simulink model "AXU5EV_Motor_Control_System"  (R2026b)
settings: Solver=FixedStepDiscrete  StopTime=0.1
model workspace (MAT data in the model file):
  ADC_Calibration_Log2_N = 10
  ADC_Manual_Offset_Valid_A = 0
  ADC_Manual_Offset_Valid_B = 0
  Angle_Init_EN : Simulink.Signal (value not decoded)
  Encoder_Counts_Per_Electrical_Period = 30000
  Encoder_Nanometres_Per_Count = 1000
  Experiment_Id_Limit_A = 0.5
  Experiment_Iq_Limit_A = 0.3
  Experiment_Parameter_Version = 20261117
  FOC_Fixed_Config : object (value not decoded)
  FOC_Fixed_Parameters : object (value not decoded)
  Feedback_Id_Step = 500
  Feedback_Tick_Hz = 50000000
  Feedback_Tick_Step = 5000
  Grating_Resolution_mm_per_count = 0.001
  Hardware_Binding_Complete = 0
  Hold_Ticks = 30000
  Host_AutoStart_EN = 0
  Host_Load_N = 0
  Host_Ready_Ticks = 5
  Host_Speed_Ramp_s = 0.2
  Host_Start_s = 0.05
  Host_Traj_Amax = 200
  Host_Traj_Jmax = 1000
  Host_Traj_Vmax = 20
  Id_Init_Step = 5e-05
  Id_Init_Target = 0.5
  Id_Release_Ramp_Ticks = 2000
  Init_Done : Simulink.Signal (value not decoded)
  Init_State_Num : Simulink.Signal (value not decoded)
  Iq_fric_run = 0.05
  Iq_fric_start = 0.4
  Iq_int_limit = 0.2
  Kaw_d = 0.0122881355932
  Kaw_q = 0.0122881355932
  Kaw_s = 0.4
  Ki_ACR = 7250
  Ki_ASR = 0.05
  Kp_ACR = 59
  Kp_ASR = 0.03
  Kp_pos = 5
  PMLSM_Kf_peak_N_per_Apeak = 21.4960461481
  PMLSM_Ld_H = 0.0118
  PMLSM_Lq_H = 0.0118
  PMLSM_Rs_ohm = 1.45
  PMLSM_psi_f_Wb = 0.0684240400279
  PMLSM_tau_NN_m = 0.03
  Physical_Calibration_Valid = 0
  Pos_deadband = 0.02
  Ramp_Ticks = 10000
  Speed_loop_Iq_Limit = 0.3
  Tau_e_mm = 30
  Theta_Offset_Fine = 0
  Theta_Offset_auto : Simulink.Signal (value not decoded)
  Total_Moving_Mass_Known = 0
  Total_Moving_Mass_kg = nan
  Ts = 0.0001
  Ts_ACR = 0.0001
  Ts_ASR = 0.001
  Ts_POS = 0.01
  Tuning_Current_Xi = 0.707106781187
  Udc = 48
  V_meas_max = 500
  V_pos_max_mmps = 20
  X_max_hard = 120
  X_max_soft = 110
  X_min_hard = -120
  X_min_soft = -110
  delay_N = 50
  id_init_ref : Simulink.Signal (value not decoded)
  theta_align_const = 0
  v_ff_eps = 0.5
  v_meas_zero_eps = 0.5
  v_over_eps = 3
  v_ref_max = 20
  v_ref_set_rate_dn = 100
  v_ref_set_rate_up = 100
  v_ref_set_step_dn = 0.01
  v_ref_set_step_up = 0.01
  v_ref_zero_eps = 0
  x_align_mm_latch : Simulink.Signal (value not decoded)
undefined symbols (not defined in the file): v_stick_off, v_stick_on
libraries: simulink x8
(part 2 of 2)

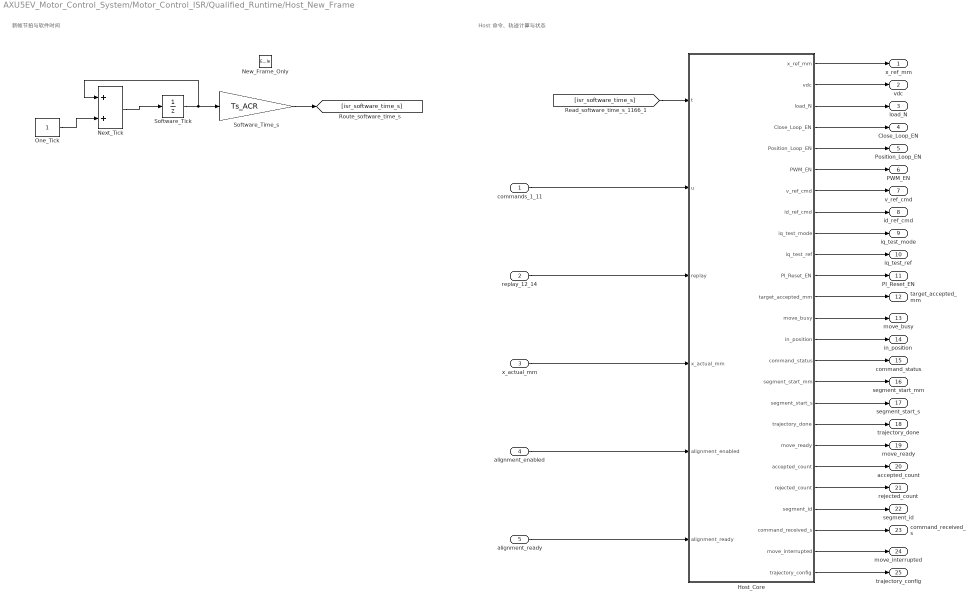
== system AXU5EV_Motor_Control_System/Motor_Control_ISR/Qualified_Runtime/Host_New_Frame ==
  note: 新帧节拍与软件时间
  note: Host 命令、轨迹计算与状态
  commands_1_11 : Inport
  replay_12_14 : Inport  Port=2
  x_actual_mm : Inport  Port=3
  alignment_enabled : Inport  Port=4
  alignment_ready : Inport  Port=5
  New_Frame_Only : EnablePort
  Host_Core : MATLAB Function  TreatAsAtomicUnit=on
  Next_Tick : Sum
  One_Tick : Constant  SampleTime=-1
  Software_Tick : UnitDelay  SampleTime=-1
  Software_Time_s : Gain  Gain=Ts_ACR
  x_ref_mm : Outport
  vdc : Outport  Port=2
  load_N : Outport  Port=3
  Close_Loop_EN : Outport  Port=4
  Position_Loop_EN : Outport  Port=5
  PWM_EN : Outport  Port=6
  v_ref_cmd : Outport  Port=7
  id_ref_cmd : Outport  Port=8
  iq_test_mode : Outport  Port=9
  iq_test_ref : Outport  Port=10
  PI_Reset_EN : Outport  Port=11
  target_accepted_mm : Outport  Port=12
  move_busy : Outport  Port=13
  in_position : Outport  Port=14
  command_status : Outport  Port=15
  segment_start_mm : Outport  Port=16
  segment_start_s : Outport  Port=17
  trajectory_done : Outport  Port=18
  move_ready : Outport  Port=19
  accepted_count : Outport  Port=20
  rejected_count : Outport  Port=21
  segment_id : Outport  Port=22
  command_received_s : Outport  Port=23
  move_interrupted : Outport  Port=24
  trajectory_config : Outport  Port=25
  wires:
  Host_Core/24(move_interrupted) -> move_interrupted/1
  Host_Core/23(command_received_s) -> command_received_s/1
  Host_Core/19(move_ready) -> move_ready/1
  Host_Core/18(trajectory_done) -> trajectory_done/1
  Host_Core/21(rejected_count) -> rejected_count/1
  x_actual_mm/1 -> Host_Core/4(x_actual_mm)
  Host_Core/22(segment_id) -> segment_id/1
  Host_Core/14(in_position) -> in_position/1
  Host_Core/13(move_busy) -> move_busy/1
  alignment_enabled/1 -> Host_Core/5(alignment_enabled)
  Host_Core/12(target_accepted_mm) -> target_accepted_mm/1
  Host_Core/9(iq_test_mode) -> iq_test_mode/1
  replay_12_14/1 -> Host_Core/3(replay)
  Host_Core/11(PI_Reset_EN) -> PI_Reset_EN/1
  Host_Core/7(v_ref_cmd) -> v_ref_cmd/1
  commands_1_11/1 -> Host_Core/2(u)
  Host_Core/10(iq_test_ref) -> iq_test_ref/1
  Host_Core/6(PWM_EN) -> PWM_EN/1
  Host_Core/5(Position_Loop_EN) -> Position_Loop_EN/1
  Host_Core/4(Close_Loop_EN) -> Close_Loop_EN/1
  Host_Core/8(id_ref_cmd) -> id_ref_cmd/1
  Host_Core/16(segment_start_mm) -> segment_start_mm/1
  One_Tick/1 -> Next_Tick/2
  Host_Core/1(x_ref_mm) -> x_ref_mm/1
  Next_Tick/1 -> Software_Tick/1
  Host_Core/3(load_N) -> load_N/1
  Host_Core/25(trajectory_config) -> trajectory_config/1
  Host_Core/17(segment_start_s) -> segment_start_s/1
  Host_Core/15(command_status) -> command_status/1
  Host_Core/20(accepted_count) -> accepted_count/1
  Host_Core/2(vdc) -> vdc/1
  alignment_ready/1 -> Host_Core/6(alignment_ready)
  Software_Tick/1 -> Software_Time_s/1, Next_Tick/1
  [isr_software_time_s] -> Host_Core/1(t)
  Software_Time_s/1 -> [isr_software_time_s]

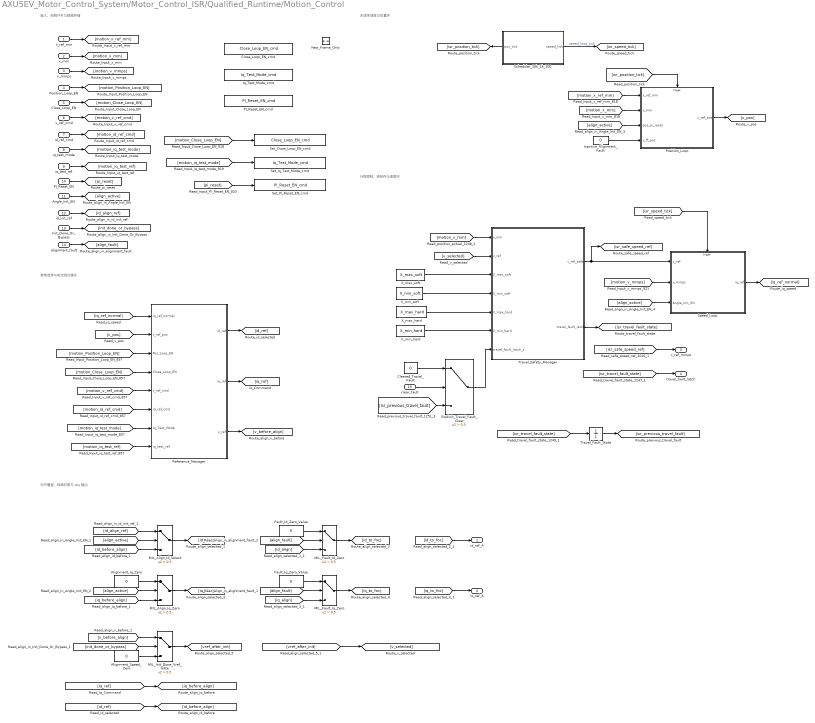
== system AXU5EV_Motor_Control_System/Motor_Control_ISR/Qualified_Runtime/Motion_Control ==
  note: 输入、控制许可与数据存储
  note: 多速率调度与位置环
  note: 参考选择与电流测试模式
  note: 行程限制、清锁存与速度环
  note: 对齐覆盖、故障归零与 d/q 输出
  x_ref_mm : Inport
  x_mm : Inport  Port=2
  v_mmps : Inport  Port=3
  Position_Loop_EN : Inport  Port=4
  Close_Loop_EN : Inport  Port=5
  v_ref_cmd : Inport  Port=6
  id_ref_cmd : Inport  Port=7
  iq_test_mode : Inport  Port=8
  iq_test_ref : Inport  Port=9
  PI_Reset_EN : Inport  Port=10
  Angle_Init_EN : Inport  Port=11
  id_init_ref : Inport  Port=12
  Init_Done_Or_Bypass : Inport  Port=13
  alignment_fault : Inport  Port=14
  clear_fault : Inport  Port=15  OutDataTypeStr=boolean  PortDimensions=1
  New_Frame_Only : EnablePort
  Alignment_Iq_Zero : Constant  Value=0  OutDataTypeStr=double
  Alignment_Speed_Zero : Constant  Value=0  OutDataTypeStr=double
  Cleared_Travel_Fault : Constant  Value=0  OutDataTypeStr=double
  Close_Loop_EN_cmd : DataStoreMemory  DataStoreName=Close_Loop_EN_cmd  WriteAfterWriteMsg=warning  InitialValue=1  ShowAdditionalParam=off
  Explicit_Travel_Fault_Clear : Switch  Criteria=u2 > Threshold  Threshold=0.5  SaturateOnIntegerOverflow=off  InputSameDT=off
  Fault_Id_Zero_Value : Constant  Value=0  OutDataTypeStr=double
  Fault_Iq_Zero_Value : Constant  Value=0  OutDataTypeStr=double
  Inactive_Alignment_Fault : Constant  Value=0
  Iq_Test_Mode_cmd : DataStoreMemory  DataStoreName=Iq_Test_Mode_cmd  WriteAfterWriteMsg=warning  ShowAdditionalParam=off
  MIL_Align_Id_Select : Switch  Criteria=u2 > Threshold  Threshold=0.5  SaturateOnIntegerOverflow=off  InputSameDT=off
  MIL_Align_Iq_Zero : Switch  Criteria=u2 > Threshold  Threshold=0.5  SaturateOnIntegerOverflow=off  InputSameDT=off
  MIL_Fault_Id_Zero : Switch  Criteria=u2 > Threshold  Threshold=0.5  SaturateOnIntegerOverflow=off  InputSameDT=off
  MIL_Fault_Iq_Zero : Switch  Criteria=u2 > Threshold  Threshold=0.5  SaturateOnIntegerOverflow=off  InputSameDT=off
  MIL_Init_Done_Vref_Gate : Switch  Criteria=u2 > Threshold  Threshold=0.5  SaturateOnIntegerOverflow=off  InputSameDT=off
  PI_Reset_EN_cmd : DataStoreMemory  DataStoreName=PI_Reset_EN_cmd  WriteAfterWriteMsg=warning  ShowAdditionalParam=off
  Position_Loop : Subsystem  TreatAsAtomicUnit=on
  Reference_Manager : Subsystem
  Scheduler_10k_1k_100 : Subsystem
      settings: PortSchema="{\"entries\":[{\"content\":{\"sides\":[{\"content\":{\"connectorIds\":[\"Out2\"]},\"type\":\"ConnectorPlacement.EquallySpacedRectSide\",\"uuid\":\"7a2cd2ad-1b6d-4ced-b4c0-dea2e76e4441\"},{\"content\":{\"connectorIds\":[\"Out1\"],\"side\":\"RIGHT\"},\"type\":\"ConnectorPlacement.EquallySpacedRectSide\",\"uuid\":\"f7db3b94-1126-4089-83bd-8e57d20e6fd7\"},{\"content\":{\"side\":\"TOP\"},\"type\":\"ConnectorPlacement.EquallySpacedRectSide\",\"uuid\":\"9153f6b5-22af-48be-92c0-68be43f93648\"}]},\"type\":\"ConnectorPlacement.EquallySpacedConnector\",\"uuid\":\"029fb485-bddc-4cd2-9c64-7547c8dffd2b\"}],\"packageUris\":[\"http://schema.mathworks.com/mf0/Connector/R2020b\"],\"version\":\"1.0\"}"
  Set_Close_Loop_EN_cmd : DataStoreWrite  Priority=-10  DataStoreName=Close_Loop_EN_cmd  IndexOptions=Index vector (dialog)  Indices=1  OutputSizes=1
  Set_Iq_Test_Mode_cmd : DataStoreWrite  Priority=-10  DataStoreName=Iq_Test_Mode_cmd  IndexOptions=Index vector (dialog)  Indices=1  OutputSizes=1
  Set_PI_Reset_EN_cmd : DataStoreWrite  Priority=-10  DataStoreName=PI_Reset_EN_cmd  IndexOptions=Index vector (dialog)  Indices=1  OutputSizes=1
  Speed_Loop : Subsystem  TreatAsAtomicUnit=on
  Travel_Fault_State : UnitDelay  SampleTime=-1
  Travel_Safety_Manager : MATLAB Function  Description=Soft +/-110 mm acts on the final speed reference before Speed_Loop and permits inward motion. Direct Iq test does not share this soft-speed limiting path. Hard +/-120 mm inclusive latches until qualified explicit clear. Mechanical encoder origin is independent of the electrical alignment offset.  TreatAsAtomicUnit=on
  X_max_hard : Constant  Value=X_max_hard  OutDataTypeStr=double
  X_max_soft : Constant  Value=X_max_soft  OutDataTypeStr=double
  X_min_hard : Constant  Value=X_min_hard  OutDataTypeStr=double
  X_min_soft : Constant  Value=X_min_soft  OutDataTypeStr=double
  id_ref_A : Outport
  iq_ref_A : Outport  Port=2
  v_ref_mmps : Outport  Port=3
  travel_fault_latch : Outport  Port=4  OutDataTypeStr=double  PortDimensions=1
  wires:
  [iq_to_foc] -> iq_ref_A/1
  [id_to_foc] -> id_ref_A/1
  [iq_ref_normal] -> Reference_Manager/1(iq_ref_normal)
  [v_pos] -> Reference_Manager/2(v_ref_pos)
  Inactive_Alignment_Fault/1 -> Position_Loop/4(v_ff_pos)
  Position_Loop/1(v_ref_pos) -> [v_pos]
  Reference_Manager/1(id_ref) -> [id_ref]
  Reference_Manager/2(iq_ref) -> [iq_ref]
  MIL_Align_Id_Select/1 -> [id_align]
  [id_align] -> MIL_Fault_Id_Zero/3
  MIL_Fault_Id_Zero/1 -> [id_to_foc]
  MIL_Align_Iq_Zero/1 -> [iq_align]
  [iq_align] -> MIL_Fault_Iq_Zero/3
  MIL_Fault_Iq_Zero/1 -> [iq_to_foc]
  [vref_after_init] -> [v_selected]
  Angle_Init_EN/1 -> [align_active]
  [align_active] -> Position_Loop/3(pos_pi_reset)
  id_init_ref/1 -> [id_align_ref]
  Init_Done_Or_Bypass/1 -> [init_done_or_bypass]
  alignment_fault/1 -> [align_fault]
  [align_fault] -> MIL_Fault_Iq_Zero/2
  [align_fault] -> MIL_Fault_Id_Zero/2
  [id_ref] -> [id_before_align]
  [id_before_align] -> MIL_Align_Id_Select/3
  [iq_ref] -> [iq_before_align]
  [iq_before_align] -> MIL_Align_Iq_Zero/3
  Reference_Manager/3(v_ref) -> [v_before_align]
  [pi_reset] -> Set_PI_Reset_EN_cmd/1
  iq_test_ref/1 -> [motion_iq_test_ref]
  [motion_iq_test_ref] -> Reference_Manager/8(iq_test_ref)
  iq_test_mode/1 -> [motion_iq_test_mode]
  [motion_iq_test_mode] -> Reference_Manager/7(Iq_Test_Mode)
  [motion_iq_test_mode] -> Set_Iq_Test_Mode_cmd/1
  id_ref_cmd/1 -> [motion_id_ref_cmd]
  [motion_id_ref_cmd] -> Reference_Manager/6(id_ref_cmd)
  v_ref_cmd/1 -> [motion_v_ref_cmd]
  [motion_v_ref_cmd] -> Reference_Manager/5(v_ref_cmd)
  Close_Loop_EN/1 -> [motion_Close_Loop_EN]
  [motion_Close_Loop_EN] -> Reference_Manager/4(Close_Loop_EN)
  [motion_Close_Loop_EN] -> Set_Close_Loop_EN_cmd/1
  Position_Loop_EN/1 -> [motion_Position_Loop_EN]
  [motion_Position_Loop_EN] -> Reference_Manager/3(Pos_Loop_EN)
  v_mmps/1 -> [motion_v_mmps]
  [motion_x_mm] -> Position_Loop/2(x_mm)
  x_ref_mm/1 -> [motion_x_ref_mm]
  [motion_x_ref_mm] -> Position_Loop/1(x_ref_mm)
  PI_Reset_EN/1 -> [pi_reset]
  [motion_v_mmps] -> Speed_Loop/2(v_mmps)
  [v_before_align] -> MIL_Init_Done_Vref_Gate/1
  [align_active] -> Speed_Loop/3(Angle_Init_EN)
  MIL_Init_Done_Vref_Gate/1 -> [vref_after_init]
  Speed_Loop/1(iq_ref) -> [iq_ref_normal]
  [isr_previous_travel_fault] -> Explicit_Travel_Fault_Clear/3
  [isr_travel_fault_state] -> Travel_Fault_State/1
  [isr_travel_fault_state] -> travel_fault_latch/1
  [isr_safe_speed_ref] -> v_ref_mmps/1
  [motion_x_mm] -> Travel_Safety_Manager/1(x_mm)
  [v_selected] -> Travel_Safety_Manager/2(v_ref)
  x_mm/1 -> [motion_x_mm]
  Cleared_Travel_Fault/1 -> Explicit_Travel_Fault_Clear/1
  clear_fault/1 -> Explicit_Travel_Fault_Clear/2
  Travel_Fault_State/1 -> [isr_previous_travel_fault]
  X_max_soft/1 -> Travel_Safety_Manager/3(X_max_soft)
  X_min_soft/1 -> Travel_Safety_Manager/4(X_min_soft)
  X_max_hard/1 -> Travel_Safety_Manager/5(X_max_hard)
  X_min_hard/1 -> Travel_Safety_Manager/6(X_min_hard)
  Explicit_Travel_Fault_Clear/1 -> Travel_Safety_Manager/7(travel_fault_latch_z)
  Travel_Safety_Manager/1(v_ref_safe) -> [isr_safe_speed_ref], Speed_Loop/1(v_ref)
  Travel_Safety_Manager/2(travel_fault_latch) -> [isr_travel_fault_state]
  [isr_speed_tick] -> Speed_Loop/Trigger
  Scheduler_10k_1k_100/1(speed_tick) -> [isr_speed_tick]  "speed_loop_tick"
  [isr_position_tick] -> Position_Loop/Trigger
  Scheduler_10k_1k_100/2(pos_tick) -> [isr_position_tick]
  Alignment_Speed_Zero/1 -> MIL_Init_Done_Vref_Gate/3
  Fault_Id_Zero_Value/1 -> MIL_Fault_Id_Zero/1
  Fault_Iq_Zero_Value/1 -> MIL_Fault_Iq_Zero/1
  Alignment_Iq_Zero/1 -> MIL_Align_Iq_Zero/1
  [init_done_or_bypass] -> MIL_Init_Done_Vref_Gate/2
  [id_align_ref] -> MIL_Align_Id_Select/1
  [align_active] -> MIL_Align_Iq_Zero/2
  [align_active] -> MIL_Align_Id_Select/2

== system AXU5EV_Motor_Control_System/Motor_Control_ISR/Qualified_Runtime/Alignment_Task/Enabled_Original_MIL ==
  note: 五态状态机与输入输出
  Init_Start : Inport
  Init_Reset : Inport  Port=2
  travel_fault_latch : Inport  Port=3
  x_mm : Inport  Port=4
  Alignment_Permit : Inport  Port=5  OutDataTypeStr=boolean
  Angle_Init : Stateflow chart  TreatAsAtomicUnit=on
  Init_Done : Outport
  Init_State_Num : Outport  Port=2
  id_init_ref : Outport  Port=3
  Angle_Init_EN : Outport  Port=4
  Theta_Offset_auto : Outport  Port=5
  x_align_mm_latch : Outport  Port=6
  wires:
  Angle_Init/4(Angle_Init_EN) -> Angle_Init_EN/1  "Angle_Init_EN"
  Angle_Init/5(Theta_Offset_auto) -> Theta_Offset_auto/1  "Theta_Offset_auto"
  Angle_Init/6(x_align_mm_latch) -> x_align_mm_latch/1  "x_align_mm_latch"
  Angle_Init/3(id_init_ref) -> id_init_ref/1  "id_init_ref"
  Angle_Init/2(Init_State_Num) -> Init_State_Num/1  "Init_State_Num"
  Angle_Init/1(Init_Done) -> Init_Done/1  "Init_Done"
  travel_fault_latch/1 -> Angle_Init/3(travel_fault_latch)
  Init_Reset/1 -> Angle_Init/2(Init_Reset)
  Init_Start/1 -> Angle_Init/1(Init_Start)
  Alignment_Permit/1 -> Angle_Init/5(Alignment_Permit)
  x_mm/1 -> Angle_Init/4(x_mm)

== system AXU5EV_Motor_Control_System/Motor_Control_ISR/Qualified_Runtime/Motion_Control/Position_Loop ==
  note: 位置误差、比例与速度前馈
  x_ref_mm : Inport
  x_mm : Inport  Port=2
  pos_pi_reset : Inport  Port=3
  v_ff_pos : Inport  Port=4
  Trigger : TriggerPort  VariantControl=(inherit)  SampleTime=-1
  Dead Zone : DeadZone  LowerValue=-Pos_deadband  UpperValue=+Pos_deadband
  Gain : Gain  Gain=Kp_pos
  Saturation : Saturate  UpperLimit=V_pos_max_mmps  LowerLimit=-V_pos_max_mmps
  Sum : Sum  Inputs=|+-
  Sum1 : Sum  Inputs=|++
  Terminator : Terminator
  v_ref_pos : Outport
  wires:
  Saturation/1 -> v_ref_pos/1  "obs_v_ref_pos"
  pos_pi_reset/1 -> Terminator/1
  Sum1/1 -> Saturation/1
  v_ff_pos/1 -> Sum1/2
  Gain/1 -> Sum1/1
  Dead Zone/1 -> Gain/1
  Sum/1 -> Dead Zone/1  "e_pos"
  x_mm/1 -> Sum/2
  x_ref_mm/1 -> Sum/1

== system AXU5EV_Motor_Control_System/Motor_Control_ISR/Qualified_Runtime/Motion_Control/Reference_Manager ==
  note: q 轴测试覆盖与 d 轴参考
  note: 速度参考选择、斜率与限幅
  iq_ref_normal : Inport
  v_ref_pos : Inport  Port=2
  Pos_Loop_EN : Inport  Port=3
  Close_Loop_EN : Inport  Port=4
  v_ref_cmd : Inport  Port=5
  id_ref_cmd : Inport  Port=6
  Iq_Test_Mode : Inport  Port=7
  iq_test_ref : Inport  Port=8
  Constant15 : Constant  Value=0
  Saturation : Saturate  UpperLimit=v_ref_max  LowerLimit=-v_ref_max
  Switch : Switch  Criteria=u2 > Threshold  Threshold=0.5  SaturateOnIntegerOverflow=off  InputSameDT=off
  Switch9 : Switch  Criteria=u2 > Threshold  Threshold=0.5  SaturateOnIntegerOverflow=off  InputSameDT=off
  v_ref_closed_sel : Switch  Criteria=u2 > Threshold  Threshold=0.5  SaturateOnIntegerOverflow=off  InputSameDT=off
  v_ref_set_slew_limiter : Subsystem
  id_ref : Outport
  iq_ref : Outport  Port=2
  v_ref : Outport  Port=3
  wires:
  v_ref_cmd/1 -> v_ref_closed_sel/3
  Saturation/1 -> Switch9/1
  Pos_Loop_EN/1 -> v_ref_closed_sel/2
  v_ref_closed_sel/1 -> v_ref_set_slew_limiter/1(v_ref_set)  "v_ref_closed"
  v_ref_pos/1 -> v_ref_closed_sel/1
  v_ref_set_slew_limiter/1(v_ref_set_limited) -> Saturation/1
  id_ref_cmd/1 -> id_ref/1
  iq_ref_normal/1 -> Switch/3
  Constant15/1 -> Switch9/3
  Iq_Test_Mode/1 -> Switch/2
  iq_test_ref/1 -> Switch/1
  Close_Loop_EN/1 -> Switch9/2
  Switch9/1 -> v_ref/1
  Switch/1 -> iq_ref/1

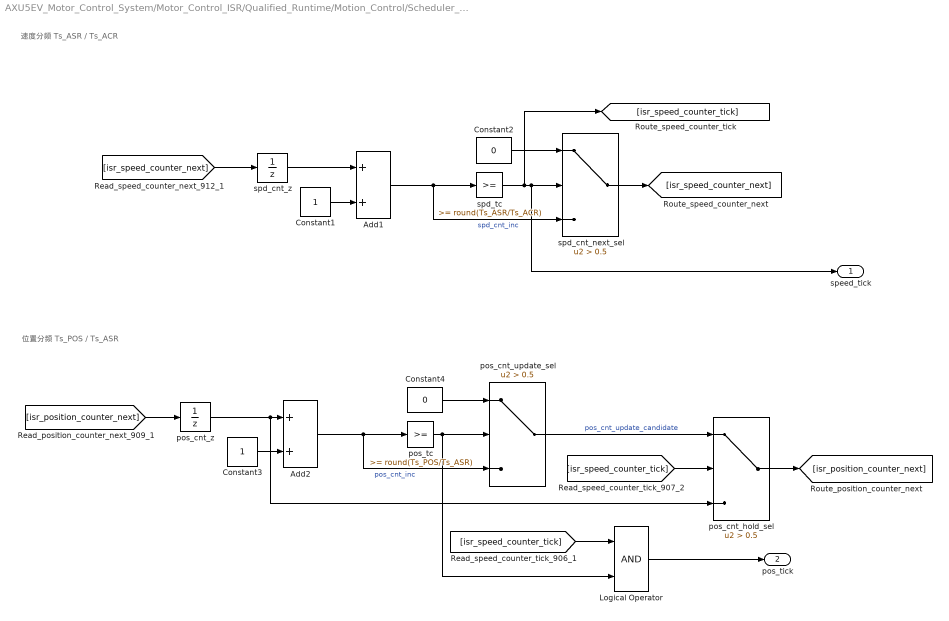
== system AXU5EV_Motor_Control_System/Motor_Control_ISR/Qualified_Runtime/Motion_Control/Scheduler_10k_1k_100 ==
  note: 速度分频 Ts_ASR / Ts_ACR
  note: 位置分频 Ts_POS / Ts_ASR
  Add1 : Sum
  Add2 : Sum
  Constant1 : Constant
  Constant2 : Constant  Value=0
  Constant3 : Constant
  Constant4 : Constant  Value=0
  Logical Operator : Logic  AllPortsSameDT=off  OutDataTypeStr=boolean
  pos_cnt_hold_sel : Switch  Criteria=u2 > Threshold  Threshold=0.5  SaturateOnIntegerOverflow=off  InputSameDT=off
  pos_cnt_update_sel : Switch  Criteria=u2 > Threshold  Threshold=0.5  SaturateOnIntegerOverflow=off  InputSameDT=off
  pos_cnt_z : UnitDelay  SampleTime=-1
  pos_tc : simulink/Logic and Bit Operations/Compare To Constant  relop=>=  const=round(Ts_POS/Ts_ASR)  OutDataTypeStr=boolean
  spd_cnt_next_sel : Switch  Criteria=u2 > Threshold  Threshold=0.5  SaturateOnIntegerOverflow=off  InputSameDT=off
  spd_cnt_z : UnitDelay  SampleTime=-1
  spd_tc : simulink/Logic and Bit Operations/Compare To Constant  relop=>=  const=round(Ts_ASR/Ts_ACR)  OutDataTypeStr=boolean
  speed_tick : Outport
  pos_tick : Outport  Port=2
  wires:
  Constant2/1 -> spd_cnt_next_sel/1
  spd_tc/1 -> speed_tick/1, spd_cnt_next_sel/2, [isr_speed_counter_tick]
  Add2/1 -> pos_cnt_update_sel/3, pos_tc/1  "pos_cnt_inc"
  [isr_position_counter_next] -> pos_cnt_z/1
  [isr_speed_counter_next] -> spd_cnt_z/1
  pos_cnt_hold_sel/1 -> [isr_position_counter_next]
  pos_cnt_update_sel/1 -> pos_cnt_hold_sel/1  "pos_cnt_update_candidate"
  Constant4/1 -> pos_cnt_update_sel/1
  pos_tc/1 -> pos_cnt_update_sel/2, Logical Operator/2
  pos_cnt_z/1 -> pos_cnt_hold_sel/3, Add2/1
  [isr_speed_counter_tick] -> Logical Operator/1
  [isr_speed_counter_tick] -> pos_cnt_hold_sel/2
  spd_cnt_z/1 -> Add1/1
  Constant1/1 -> Add1/2
  spd_cnt_next_sel/1 -> [isr_speed_counter_next]
  Add1/1 -> spd_cnt_next_sel/3, spd_tc/1  "spd_cnt_inc"
  Constant3/1 -> Add2/2
  Logical Operator/1 -> pos_tick/1

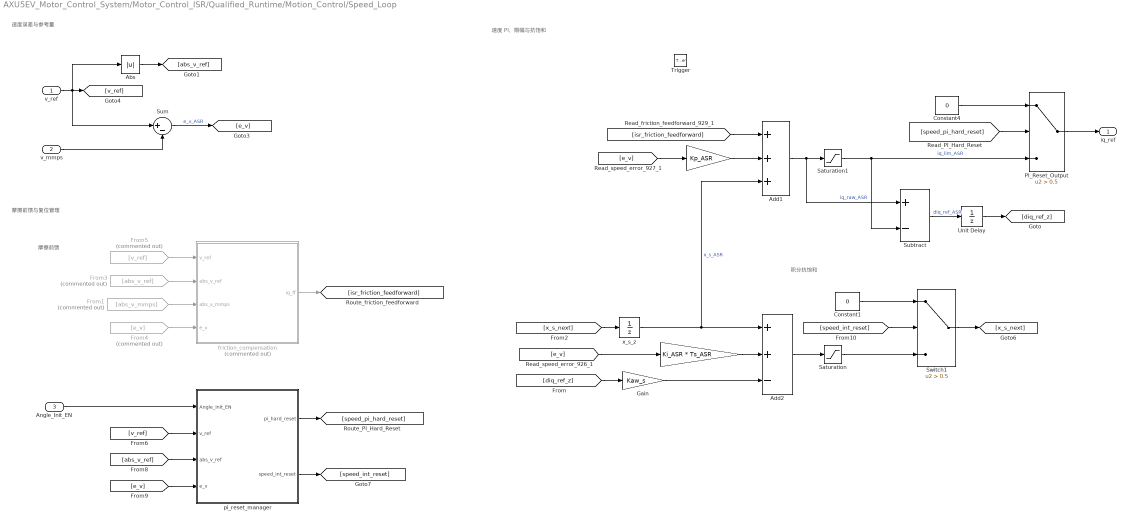
== system AXU5EV_Motor_Control_System/Motor_Control_ISR/Qualified_Runtime/Motion_Control/Speed_Loop ==
  note: 摩擦前馈
  note: 积分抗饱和
  note: 速度误差与参考量
  note: 摩擦前馈与复位管理
  note: 速度 PI、限幅与抗饱和
  v_ref : Inport
  v_mmps : Inport  Port=2
  Angle_Init_EN : Inport  Port=3
  Trigger : TriggerPort  VariantControl=(inherit)  SampleTime=-1
  " " : Gain  Gain=Ki_ASR * Ts_ASR
  "  " : Gain  Gain=Kp_ASR
  Abs : Abs  SaturateOnIntegerOverflow=off
  Add1 : Sum  Inputs=+++
  Add2 : Sum  Inputs=++-
  Constant1 : Constant  Value=0
  Constant4 : Constant  Value=0
  From1 : From  Commented=on  GotoTag=abs_v_mmps
  From3 : From  Commented=on  GotoTag=abs_v_ref
  From4 : From  Commented=on  GotoTag=e_v
  From5 : From  Commented=on  GotoTag=v_ref
  Gain : Gain  Gain=Kaw_s
  PI_Reset_Output : Switch  Criteria=u2 > Threshold  Threshold=0.5  SaturateOnIntegerOverflow=off  InputSameDT=off
  Saturation : Saturate  UpperLimit=Iq_int_limit  LowerLimit=-Iq_int_limit
  Saturation1 : Saturate  UpperLimit=Speed_loop_Iq_Limit  LowerLimit=-Speed_loop_Iq_Limit
  Subtract : Sum  Inputs=+-
  Sum : Sum  Inputs=|+-
  Switch1 : Switch  Criteria=u2 > Threshold  Threshold=0.5  SaturateOnIntegerOverflow=off  InputSameDT=off
  Unit Delay : UnitDelay  SampleTime=-1
  friction_compensation : Subsystem  Commented=on
  pi_reset_manager : Subsystem
  x_s_z : UnitDelay  SampleTime=-1
  iq_ref : Outport
  wires:
  Saturation/1 -> Switch1/3
  Switch1/1 -> [x_s_next]
  [speed_int_reset] -> Switch1/2
  pi_reset_manager/1(pi_hard_reset) -> [speed_pi_hard_reset]
  pi_reset_manager/2(speed_int_reset) -> [speed_int_reset]
  [speed_pi_hard_reset] -> PI_Reset_Output/2
  [e_v] -> pi_reset_manager/4(e_v)
  [abs_v_ref] -> pi_reset_manager/3(abs_v_ref)
  [v_ref] -> pi_reset_manager/2(v_ref)
  From5/1 -> friction_compensation/1(v_ref)
  Angle_Init_EN/1 -> pi_reset_manager/1(Angle_Init_EN)
  Abs/1 -> [abs_v_ref]
  From3/1 -> friction_compensation/2(abs_v_ref)
  From1/1 -> friction_compensation/3(abs_v_mmps)
  From4/1 -> friction_compensation/4(e_v)
  Constant4/1 -> PI_Reset_Output/1
  PI_Reset_Output/1 -> iq_ref/1
  Constant1/1 -> Switch1/1
  [diq_ref_z] -> Gain/1
  Unit Delay/1 -> [diq_ref_z]
  Subtract/1 -> Unit Delay/1  "diq_ref_ASR"
  [x_s_next] -> x_s_z/1
  Saturation1/1 -> Subtract/2, PI_Reset_Output/3  "iq_lim_ASR"
  [isr_friction_feedforward] -> Add1/1
  [e_v] -> "  "/1
  [e_v] -> " "/1
  Sum/1 -> [e_v]  "e_v_ASR"
  Add1/1 -> Subtract/1, Saturation1/1  "iq_raw_ASR"
  v_ref/1 -> [v_ref], Sum/1, Abs/1
  Add2/1 -> Saturation/1
  Gain/1 -> Add2/3
  " "/1 -> Add2/2
  "  "/1 -> Add1/2
  friction_compensation/1(iq_ff) -> [isr_friction_feedforward]
  x_s_z/1 -> Add1/3, Add2/1  "x_s_ASR"
  v_mmps/1 -> Sum/2

== system AXU5EV_Motor_Control_System/Motor_Control_ISR/Qualified_Runtime/Motion_Control/Reference_Manager/v_ref_set_slew_limiter ==
  note: 速度参考变化量与离散保持
  v_ref_set : Inport
  Add : Sum
  Saturation : Saturate  UpperLimit=v_ref_set_step_up  LowerLimit=-v_ref_set_step_dn
  Subtract : Sum  Inputs=+-
  v_ref_set_lim_z : UnitDelay  SampleTime=-1
  v_ref_set_limited : Outport
  wires:
  Add/1 -> v_ref_set_lim_z/1, v_ref_set_limited/1
  Subtract/1 -> Saturation/1
  Saturation/1 -> Add/1
  v_ref_set/1 -> Subtract/1
  v_ref_set_lim_z/1 -> Add/2, Subtract/2

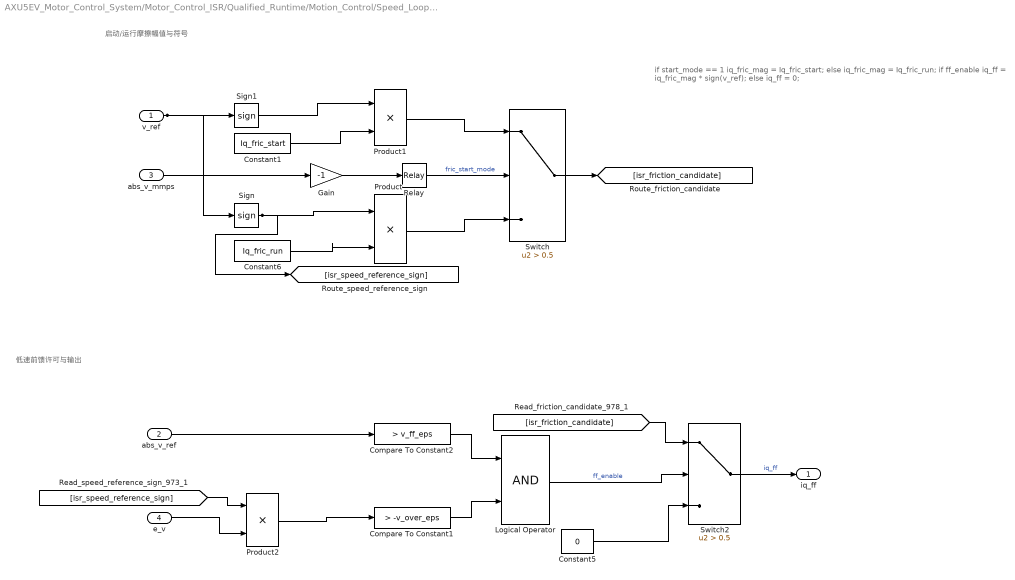
== system AXU5EV_Motor_Control_System/Motor_Control_ISR/Qualified_Runtime/Motion_Control/Speed_Loop/friction_compensation ==
  note: if start_mode == 1
      | 	iq_fric_mag = Iq_fric_start;
      | else
      | 	iq_fric_mag = Iq_fric_run;
      |
      | if ff_enable
      | 	iq_ff = iq_fric_mag * sign(v_ref);
      |  else
      | 	iq_ff = 0;
  note: 启动/运行摩擦幅值与符号
  note: 低速前馈许可与输出
  v_ref : Inport
  abs_v_ref : Inport  Port=2
  abs_v_mmps : Inport  Port=3
  e_v : Inport  Port=4
  Compare To Constant1 : simulink/Logic and Bit Operations/Compare To Constant  relop=>  const=-v_over_eps  OutDataTypeStr=boolean
  Compare To Constant2 : simulink/Logic and Bit Operations/Compare To Constant  relop=>  const=v_ff_eps  OutDataTypeStr=boolean
  Constant1 : Constant  Value=Iq_fric_start
  Constant5 : Constant  Value=0
  Constant6 : Constant  Value=Iq_fric_run
  Gain : Gain  Gain=-1
  Logical Operator : Logic  AllPortsSameDT=off  OutDataTypeStr=boolean
  Product : Product
  Product1 : Product
  Product2 : Product
  Relay : Relay  OnSwitchValue=-v_stick_on  OffSwitchValue=-v_stick_off
  Sign : Signum
  Sign1 : Signum
  Switch : Switch  Criteria=u2 > Threshold  Threshold=0.5  SaturateOnIntegerOverflow=off  InputSameDT=off
  Switch2 : Switch  Criteria=u2 > Threshold  Threshold=0.5  SaturateOnIntegerOverflow=off  InputSameDT=off
  iq_ff : Outport
  wires:
  Gain/1 -> Relay/1
  Relay/1 -> Switch/2  "fric_start_mode"
  abs_v_mmps/1 -> Gain/1
  Logical Operator/1 -> Switch2/2  "ff_enable"
  Compare To Constant1/1 -> Logical Operator/2
  Compare To Constant2/1 -> Logical Operator/1
  Product2/1 -> Compare To Constant1/1
  e_v/1 -> Product2/2
  Product1/1 -> Switch/1
  Constant1/1 -> Product1/2
  Sign1/1 -> Product1/1
  Product/1 -> Switch/3
  Switch2/1 -> iq_ff/1  "iq_ff"
  abs_v_ref/1 -> Compare To Constant2/1
  Constant6/1 -> Product/2
  Constant5/1 -> Switch2/3
  v_ref/1 -> Sign1/1, Sign/1
  [isr_speed_reference_sign] -> Product2/1
  [isr_friction_candidate] -> Switch2/1
  Sign/1 -> [isr_speed_reference_sign], Product/1
  Switch/1 -> [isr_friction_candidate]

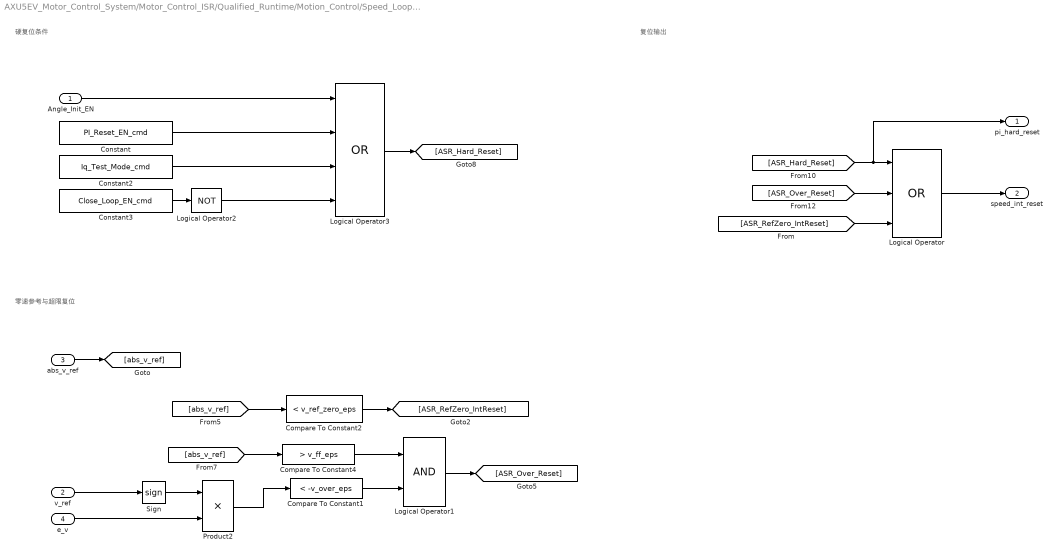
== system AXU5EV_Motor_Control_System/Motor_Control_ISR/Qualified_Runtime/Motion_Control/Speed_Loop/pi_reset_manager ==
  note: 硬复位条件
  note: 零速参考与超限复位
  note: 复位输出
  Angle_Init_EN : Inport
  v_ref : Inport  Port=2
  abs_v_ref : Inport  Port=3
  e_v : Inport  Port=4
  Compare To Constant1 : simulink/Logic and Bit Operations/Compare To Constant  relop=<  const=-v_over_eps  OutDataTypeStr=boolean
  Compare To Constant2 : simulink/Logic and Bit Operations/Compare To Constant  relop=<  const=v_ref_zero_eps  OutDataTypeStr=boolean
  Compare To Constant4 : simulink/Logic and Bit Operations/Compare To Constant  relop=>  const=v_ff_eps  OutDataTypeStr=boolean
  Constant : DataStoreRead  DataStoreName=PI_Reset_EN_cmd  IndexOptions=Index vector (dialog)  Indices=1  OutputSizes=1
  Constant2 : DataStoreRead  DataStoreName=Iq_Test_Mode_cmd  IndexOptions=Index vector (dialog)  Indices=1  OutputSizes=1
  Constant3 : DataStoreRead  DataStoreName=Close_Loop_EN_cmd  IndexOptions=Index vector (dialog)  Indices=1  OutputSizes=1
  Logical Operator : Logic  Operator=OR  Inputs=3  AllPortsSameDT=off  OutDataTypeStr=boolean
  Logical Operator1 : Logic  AllPortsSameDT=off  OutDataTypeStr=boolean
  Logical Operator2 : Logic  Operator=NOT  AllPortsSameDT=off  OutDataTypeStr=boolean
  Logical Operator3 : Logic  Operator=OR  Inputs=4  AllPortsSameDT=off  OutDataTypeStr=boolean
  Product2 : Product
  Sign : Signum
  pi_hard_reset : Outport
  speed_int_reset : Outport  Port=2
  wires:
  Constant/1 -> Logical Operator3/2
  Constant3/1 -> Logical Operator2/1
  Constant2/1 -> Logical Operator3/3
  Logical Operator2/1 -> Logical Operator3/4
  Angle_Init_EN/1 -> Logical Operator3/1
  Logical Operator3/1 -> [ASR_Hard_Reset]
  [ASR_Hard_Reset] -> Logical Operator/1, pi_hard_reset/1
  [ASR_Over_Reset] -> Logical Operator/2
  Logical Operator/1 -> speed_int_reset/1
  [ASR_RefZero_IntReset] -> Logical Operator/3
  Logical Operator1/1 -> [ASR_Over_Reset]
  abs_v_ref/1 -> [abs_v_ref]
  v_ref/1 -> Sign/1
  Compare To Constant4/1 -> Logical Operator1/1
  Compare To Constant1/1 -> Logical Operator1/2
  Product2/1 -> Compare To Constant1/1
  Sign/1 -> Product2/1
  e_v/1 -> Product2/2
  [abs_v_ref] -> Compare To Constant4/1
  [abs_v_ref] -> Compare To Constant2/1
  Compare To Constant2/1 -> [ASR_RefZero_IntReset]

== stateflow chart AXU5EV_Motor_Control_System/Motor_Control_ISR/Qualified_Runtime/Alignment_Task/Enabled_Original_MIL/Angle_Init ==
  note: 固定电角度，缓慢建立 d 轴电流。
  note: 保持固定电角度，让动子吸附稳定。
  state IDLE
    entry:
    Angle_Init_EN = 0;
    Init_Done = 0;
    id_init_ref = 0;
    Init_State_Num = 0;
    Start_Armed = ...
    (Init_Start < 0.5);
    during:
    Start_Armed = ...
    (Init_Start < 0.5);
  state RAMP_ID
    entry:
    Angle_Init_EN   = 1;
    Init_Done       = 0;
    id_init_ref     = 0;
    Init_State_Num  = 1;
    during:
    Angle_Init_EN = 1;
    Init_Done     = 0;
    id_init_ref = id_init_ref + Id_Init_Step;
    if (id_init_ref > Id_Init_Target)
    id_init_ref = Id_Init_Target;
    end
  state HOLD_ALIGN
    entry:
    Angle_Init_EN   = 1;
    Init_Done       = 0;
    id_init_ref     = Id_Init_Target;
    Init_State_Num  = 2;
    during:
    Angle_Init_EN = 1;
    Init_Done     = 0;
    id_init_ref   = Id_Init_Target;
  state RAMP_DOWN_ID
    entry:
    Angle_Init_EN   = 1;
    Init_Done       = 0;
    id_init_ref     = Id_Init_Target;
    Init_State_Num  = 3;
    during:
    Angle_Init_EN = 1;
    Init_Done     = 0;
    id_init_ref = id_init_ref - Id_Init_Target/Id_Release_Ramp_Ticks;
    if (id_init_ref < 0)
    id_init_ref = 0;
    end
    Theta_Offset_auto = theta_offset_mem;
  state DONE
    entry:
    Angle_Init_EN   = 0;
    Init_Done       = 1;
    id_init_ref     = 0;
    Init_State_Num  = 4;
    during:
    Angle_Init_EN = 0;
    Init_Done = 1;
    id_init_ref = 0;
    Init_State_Num = 4;
    Theta_Offset_auto = theta_offset_mem;
  HOLD_ALIGN -> IDLE [order 1] : [Init_Reset > 0.5 || ...
      |  travel_fault_latch > 0.5 || ...
      |  ~Alignment_Permit]
      | {theta_offset_mem = 0;
      |  Theta_Offset_auto = 0;
      |  x_align_mm_latch = 0;}
  RAMP_ID -> IDLE [order 1] : [Init_Reset > 0.5 || ...
      |  travel_fault_latch > 0.5 || ...
      |  ~Alignment_Permit]
      | {theta_offset_mem = 0;
      |  Theta_Offset_auto = 0;
      |  x_align_mm_latch = 0;}
  (default) -> IDLE
  IDLE -> RAMP_ID : [Start_Armed && Init_Start > 0.5 && ...
      |  Alignment_Permit && Init_Reset < 0.5 && ...
      |  travel_fault_latch < 0.5]
      | {Start_Armed = false;}
  RAMP_ID -> HOLD_ALIGN [order 2] : [after(Ramp_Ticks, tick)]
  RAMP_DOWN_ID -> IDLE [order 1] : [Init_Reset > 0.5 || ...
      |  travel_fault_latch > 0.5 || ...
      |  ~Alignment_Permit]
      | {theta_offset_mem = 0;
      |  Theta_Offset_auto = 0;
      |  x_align_mm_latch = 0;}
  DONE -> IDLE : [Init_Reset > 0.5 || travel_fault_latch > 0.5]
  HOLD_ALIGN -> RAMP_DOWN_ID [order 2] : [after(Hold_Ticks, tick)]
      | {x_align_mm_latch = x_mm;
      | theta_offset_mem = mod(theta_align_const - 2*pi*x_align_mm_latch/Tau_e_mm, 2*pi);
      | Theta_Offset_auto = theta_offset_mem;}
  RAMP_DOWN_ID -> DONE [order 2] : [after(Id_Release_Ramp_Ticks, tick)]
  data: Init_Start input; Init_Reset input; travel_fault_latch input; Init_Done output; Init_State_Num output; theta_align_const parameter; Tau_e_mm parameter; Id_Init_Target parameter; Ramp_Ticks parameter; Hold_Ticks parameter; Id_Init_Step parameter; id_init_ref output; Angle_Init_EN output; x_mm input; Theta_Offset_auto output; x_align_mm_latch output; theta_offset_mem local; Id_Release_Ramp_Ticks parameter; Alignment_Permit input boolean; Start_Armed local boolean

== matlab function AXU5EV_Motor_Control_System/Motor_Control_ISR/Reference_Commit ==
  data: runtime input; reference output; healthy input; speed_valid input; speed_mm_s input; sample_id input; new_frame input; request_freset input; relcon input; encon input; oe_disable input; external_fault input; travel_fault input; id_limit input; iq_limit input; tau_mm input; commit_id output; reference_version output
function [reference,commit_id,reference_version]=f( ...
    runtime,healthy,speed_valid,speed_mm_s,sample_id,new_frame,request_freset, ...
    relcon,encon,oe_disable,external_fault,travel_fault,id_limit,iq_limit,tau_mm)
%#codegen
% Atomic reference/permission adapter. The PL current loop remains external.
persistent version last_id
if isempty(version)
    version=uint32(0);
    last_id=uint32(0);
end
if new_frame
    if version==uint32(4294967295)
        version=uint32(0);
    else
        version=version+uint32(1);
    end
    last_id=sample_id;
end
runtime_finite=all(isfinite(runtime));
valid=new_frame && healthy && speed_valid && ~external_fault && ...
    travel_fault<=0.5 && runtime_finite;
pwm=valid && runtime(18)~=0 && relcon && encon && ~oe_disable && ~request_freset;
id_ref=min(id_limit,max(-id_limit,runtime(1)));
iq_ref=min(iq_limit,max(-iq_limit,runtime(2)));
if ~valid
    id_ref=0;
    iq_ref=0;
end
omega=speed_mm_s*(2*pi/tau_mm);
if ~speed_valid || ~isfinite(omega)
    omega=0;
end
pi_reset=runtime(23)~=0 || ~pwm || ~valid;
theta_offset=runtime(8);
angle_init=runtime(7);
if ~runtime_finite
    theta_offset=0;
    angle_init=0;
end
reference=[id_ref;iq_ref;omega;theta_offset;angle_init; ...
    double(pwm);double(pi_reset);double(valid)];
commit_id=last_id;
reference_version=version;
end

== matlab function AXU5EV_Motor_Control_System/Motor_Control_ISR/Capture_Latest_Observation ==
  data: sample_id input; data output; reference_version input; position_mm input; speed_mm_s input; runtime input; reference input; fault input
function data=f(sample_id,reference_version,position_mm, ...
    speed_mm_s,runtime,reference,fault)
%#codegen
% Latest complete observation, consumed by the separate service entry.
data=[double(sample_id);double(reference_version);position_mm;speed_mm_s; ...
    runtime(5);reference(1);reference(2);reference(3);reference(4); ...
    reference(6);reference(8);double(fault)];
end

== matlab function AXU5EV_Motor_Control_System/NonRealtime_Service/Count_Service_Call ==
  data: previous input; next output
function next=f(previous)
%#codegen
if previous==uint32(4294967295)
    next=uint32(0);
else
    next=previous+uint32(1);
end
end

== matlab function AXU5EV_Motor_Control_System/Motor_Control_ISR/Alignment_Permit ==
  data: command input; permit output; initialized input; position_valid input; speed_valid input; history_count input; status input; current_valid input; control_fault input; relcon input; encon input; oe_disable input; freset input; safety_process output; driver_reset output; delay_N parameter double
function [permit,safety_process,driver_reset]=f(command,initialized,position_valid,speed_valid,history_count,status,current_valid,control_fault,relcon,encon,oe_disable,freset, delay_N)
%#codegen
% Software permit only. Physical current establishment is HW_BINDING_PENDING.
% Duplicate reads keep a previously complete speed history.
duplicate = bitand(status,uint32(2))~=uint32(0);
feedback_ready = position_valid && current_valid && ...
    (speed_valid || (duplicate && history_count>=uint8(delay_N+1)));
init_reset = command(18)>0.5;
pi_reset = command(9)~=0;
permit = initialized && feedback_ready && ~control_fault && ...
    command(8)>0.5 && command(16)>0.5 && relcon && encon && ...
    ~oe_disable && ~freset && ~init_reset && ~pi_reset;
% Safety executes even when no new valid feedback frame is available.
safety_process = initialized && ~permit;
driver_reset = freset || init_reset;
end

== matlab function AXU5EV_Motor_Control_System/Motor_Control_ISR/Feedback_Measurement/Frame_And_Count_Guard ==
  data: raw_count input; continuous_count output; sample_id input; sample_tick input; encoder_ready input; illegal_count input; zero_count input; reverse input; config_version input; nm_per_count input; reset input; origin_count output; advance output; restart_history output; position_valid output; speed_valid output; history_count output; status output; Feedback_Id_Step parameter uint32; Feedback_Tick_Step parameter uint64; delay_N parameter double
function [continuous_count,origin_count,advance,restart_history,position_valid,speed_valid,history_count,status] = f(raw_count,sample_id,sample_tick,encoder_ready,illegal_count,zero_count,reverse,config_version,nm_per_count,reset, Feedback_Id_Step, Feedback_Tick_Step, delay_N)
%#codegen
% The initialization file defines the expected frame and timestamp steps.
% delay_N+1 accepted positions fill the speed history. Duplicate reads preserve
% position/count/history, report speed invalid, and do not advance the Delay.
% An integral missing-frame gap preserves continuous count and restarts the
% speed history. Invalid/restart status is handled by the upper fault latch.
% Status bit 0 startup, 1 duplicate, 2 gap, 3 config-history reset,
% 4 invalid encoder/illegal transition, 5 ambiguous half-wrap, 6 resynchronize.
% restart_history also accompanies startup/gap/config and is a separate output.
STATUS_STARTUP=uint32(1);
STATUS_DUPLICATE=uint32(2);
STATUS_GAP=uint32(4);
STATUS_CONFIG_HISTORY_RESET=uint32(8);
STATUS_INVALID_ENCODER=uint32(16);
STATUS_AMBIGUOUS_HALF_WRAP=uint32(32);
STATUS_RESTART=uint32(64);
% Frame qualification and modulo-count adaptation for the visible DSP graph.
% Position scaling, the sample-window difference and speed scaling live in SLX.
% Retains the qualified-frame behavior of encoder_position_speed.
persistent initialized last_raw last_id last_tick last_bad total origin
persistent old_zero old_reverse old_version old_scale filled
if isempty(initialized)
    initialized=false;
    last_raw=uint32(0);last_id=uint32(0);last_tick=uint64(0);last_bad=uint32(0);
    total=int64(0);origin=int64(0);old_zero=uint32(0);old_reverse=false;
    old_version=uint32(0);old_scale=uint32(0);filled=uint8(0);
end
continuous_count=total;origin_count=origin;
advance=false;restart_history=false;position_valid=false;speed_valid=false;
history_count=filled;status=uint32(0);
if reset
    initialized=false;filled=uint8(0);total=int64(0);origin=int64(0);
    continuous_count=int64(0);origin_count=int64(0);history_count=uint8(0);
    restart_history=true;
    return;
end
if ~encoder_ready || nm_per_count==0
    initialized=false;filled=uint8(0);history_count=uint8(0);
    restart_history=true;status=STATUS_INVALID_ENCODER;
    return;
end
if initialized
    id_delta=mod32diff(sample_id,last_id);
    tick_delta=mod64diff(sample_tick,last_tick);
    if id_delta==0 && tick_delta==0
        status=STATUS_DUPLICATE;position_valid=true;
        if raw_count~=last_raw || illegal_count~=last_bad
            initialized=false;filled=uint8(0);position_valid=false;
            restart_history=true;status=bitor(STATUS_DUPLICATE,bitor(STATUS_INVALID_ENCODER,STATUS_RESTART));
        end
        history_count=filled;
        return;
    end
    if illegal_count~=last_bad
        initialized=false;filled=uint8(0);history_count=uint8(0);
        restart_history=true;status=STATUS_INVALID_ENCODER;
        return;
    end
    if id_delta~=uint64(Feedback_Id_Step) || tick_delta~=Feedback_Tick_Step
        if id_delta==0 || id_delta>2147483647 || ...
                mod(id_delta,uint64(Feedback_Id_Step))~=0 || ...
                tick_delta~=id_delta*idivide(Feedback_Tick_Step,uint64(Feedback_Id_Step),'floor')
            initialized=false;filled=uint8(0);history_count=uint8(0);
            restart_history=true;status=bitor(STATUS_INVALID_ENCODER,STATUS_RESTART);
            return;
        end
        filled=uint8(0);restart_history=true;status=STATUS_GAP;
    end
    delta=count_delta(raw_count,last_raw);
    if delta==int64(-2147483648)
        initialized=false;filled=uint8(0);history_count=uint8(0);
        restart_history=true;status=bitor(STATUS_INVALID_ENCODER,STATUS_AMBIGUOUS_HALF_WRAP);
        return;
    end
    total=total+delta;
else
    total=count_delta(raw_count,uint32(0));
    status=STATUS_STARTUP;filled=uint8(0);restart_history=true;
end
changed=~initialized || zero_count~=old_zero || reverse~=old_reverse || ...
    config_version~=old_version || nm_per_count~=old_scale;
if changed
    if ~initialized || zero_count~=old_zero
        relative=count_delta(raw_count,zero_count);
        if relative==int64(-2147483648)
            initialized=false;filled=uint8(0);history_count=uint8(0);
            restart_history=true;status=bitor(STATUS_INVALID_ENCODER,STATUS_AMBIGUOUS_HALF_WRAP);
            return;
        end
        origin=total-relative;
    end
    if initialized,status=bitor(status,STATUS_CONFIG_HISTORY_RESET);end
    filled=uint8(0);restart_history=true;
end
initialized=true;last_raw=raw_count;last_id=sample_id;
last_tick=sample_tick;last_bad=illegal_count;
old_zero=zero_count;old_reverse=reverse;old_version=config_version;old_scale=nm_per_count;
history_needed=uint8(delay_N+1);
if filled<history_needed,filled=filled+uint8(1);end
continuous_count=total;origin_count=origin;advance=true;
position_valid=true;speed_valid=filled==history_needed;history_count=filled;
end

function delta=count_delta(current,previous)
delta=int64(current)-int64(previous);
if delta>int64(2147483647)
    delta=delta-int64(4294967296);
elseif delta<int64(-2147483648)
    delta=delta+int64(4294967296);
end
end

function delta=mod32diff(current,previous)
if current>=previous
    delta=uint64(current)-uint64(previous);
else
    delta=uint64(4294967296)-uint64(previous)+uint64(current);
end
end

function delta=mod64diff(current,previous)
if current>=previous
    delta=current-previous;
else
    delta=(intmax('uint64')-previous)+current+uint64(1);
end
end

== matlab function AXU5EV_Motor_Control_System/Motor_Control_ISR/Qualified_Runtime/Motion_Control/Travel_Safety_Manager ==
  data: v_ref_safe output; x_mm input; travel_fault_latch output; v_ref input; X_max_soft input; X_min_soft input; X_max_hard input; X_min_hard input; travel_fault_latch_z input
function [v_ref_safe, travel_fault_latch] = Travel_Safety_Manager( ...
    x_mm, v_ref, X_max_soft, X_min_soft, X_max_hard, X_min_hard, travel_fault_latch_z)
% PMLSM travel safety manager
% 功能：
% 1. 软限位：只限制继续向越界方向运动，不触发硬关断
% 2. 硬限位：触发 travel_fault_latch，锁存故障
% 3. travel_fault_latch = 1 后，v_ref_safe 强制为 0
% 注意：
% 上一拍锁存由外部状态块保持，明确安全清除输入控制其复位。
% PI_Reset、Init_Reset 与驱动 F_Reset 保持各自职责。
% 速度方向判断死区，单位 mm/s
V_eps = 0.0;

% ---------- 1. 硬限位检测 ----------
hard_hi = (x_mm >= X_max_hard);
hard_lo = (x_mm <= X_min_hard);
hard_fault_raw = hard_hi || hard_lo;

% ---------- 2. 外部锁存 ----------
% 上一拍已经故障，或者当前触发硬限位，则继续保持故障
fault_latch_now = (travel_fault_latch_z > 0.5) || hard_fault_raw;

% ---------- 3. 软限位方向性限制 ----------
right_soft = (x_mm >= X_max_soft);
left_soft  = (x_mm <= X_min_soft);

v_pos_dir = (v_ref >  V_eps);
v_neg_dir = (v_ref < -V_eps);

right_block = right_soft && v_pos_dir;
left_block  = left_soft  && v_neg_dir;

soft_block = right_block || left_block;

% ---------- 4. 输出安全速度 ----------
if fault_latch_now
    v_ref_safe = 0.0;
elseif soft_block
    v_ref_safe = 0.0;
else
    v_ref_safe = v_ref;
end

travel_fault_latch = double(fault_latch_now);
end

== matlab function AXU5EV_Motor_Control_System/Motor_Control_ISR/Bind_Real_Feedback/Finite_Command ==
  data: command input; clean output; pi_request output
function [clean,pi_request]=f(command)
%#codegen
clean=command;
if ~all(isfinite(command)),clean=zeros(20,1);end
pi_request=command(9)~=0;
end

== matlab function AXU5EV_Motor_Control_System/Motor_Control_ISR/Frame_And_Fault_Qualification ==
  data: initialized input; new_frame output; erri_n input; erru_n input; current_valid input; position_valid input; feedback_status input; position_mm input; command input; clear_fault input; request_freset input; max_hard input; min_hard input; healthy output; fault_latched output; clear_allowed output
function [new_frame,healthy,fault_latched,clear_allowed]=f( ...
    initialized,erri_n,erru_n,current_valid,position_valid,feedback_status, ...
    position_mm,command,clear_fault,request_freset,max_hard,min_hard)
%#codegen
% Glue between qualified feedback and the copied control/driver algorithms.
% The measurement component owns count continuity and duplicate detection.
persistent fault
if isempty(fault)
    fault=false;
end
% Measurement status bits are defined in Frame_And_Count_Guard.
% A duplicate alone preserves the count/history and does not latch a fault.
STATUS_DUPLICATE=uint32(2);
STATUS_GAP=uint32(4);
STATUS_INVALID_ENCODER=uint32(16);
STATUS_AMBIGUOUS_HALF_WRAP=uint32(32);
STATUS_RESTART=uint32(64);
bad_status_bits=bitor(STATUS_GAP,bitor(STATUS_INVALID_ENCODER, ...
    bitor(STATUS_AMBIGUOUS_HALF_WRAP,STATUS_RESTART)));
duplicate=bitand(feedback_status,STATUS_DUPLICATE)~=uint32(0);
bad_feedback=~position_valid || ~current_valid || ...
    bitand(feedback_status,bad_status_bits)~=uint32(0);
raw_fault=~erri_n || ~erru_n;
hard_fault=position_valid && (position_mm>=max_hard || position_mm<=min_hard);
command_valid=all(isfinite(command));
clear_allowed=initialized && position_valid && ~duplicate && clear_fault && ...
    ~raw_fault && ~hard_fault && ...
    ~bad_feedback && command_valid && command(8)==0;
if clear_allowed
    fault=false;
elseif raw_fault || hard_fault || bad_feedback || ~command_valid
    fault=true;
end
new_frame=initialized && position_valid && ~duplicate;
healthy=new_frame && ~fault && ~raw_fault && ~hard_fault && ...
    current_valid && command_valid && ~request_freset;
fault_latched=fault;
end

== matlab function AXU5EV_Motor_Control_System/Motor_Control_ISR/Qualified_Runtime/Host_New_Frame/Host_Core ==
  settings: sampleTime=Ts_ACR
  data: t input; u input; replay input; x_actual_mm input; alignment_enabled input; alignment_ready input; x_ref_mm output; vdc output; load_N output; Close_Loop_EN output; Position_Loop_EN output; PWM_EN output; v_ref_cmd output; id_ref_cmd output; iq_test_mode output; iq_test_ref output; PI_Reset_EN output; Host_Start_s parameter; Udc parameter; Host_Load_N parameter; Host_Traj_Vmax parameter; Host_Traj_Amax parameter; Host_Traj_Jmax parameter; Host_Speed_Ramp_s parameter; target_accepted_mm output; move_busy output; in_position output; command_status output; segment_start_mm output; segment_start_s output; trajectory_done output; move_ready output; accepted_count output; rejected_count output; segment_id output; command_received_s output; move_interrupted output; Ts_ACR parameter; Ts_POS parameter; Pos_deadband parameter; Host_Ready_Ticks parameter; Host_AutoStart_EN parameter; trajectory_config output
function [x_ref_mm,vdc,load_N,Close_Loop_EN,Position_Loop_EN,PWM_EN,v_ref_cmd,id_ref_cmd,iq_test_mode,iq_test_ref,PI_Reset_EN,target_accepted_mm,move_busy,in_position,command_status,segment_start_mm,segment_start_s,trajectory_done,move_ready,accepted_count,rejected_count,segment_id,command_received_s,move_interrupted,trajectory_config]=Simple_Host(t,u,replay,x_actual_mm,alignment_enabled,alignment_ready,Host_Start_s,Udc,Host_Load_N,Host_Traj_Vmax,Host_Traj_Amax,Host_Traj_Jmax,Host_Speed_Ramp_s,Ts_ACR, Ts_POS, Pos_deadband, Host_Ready_Ticks, Host_AutoStart_EN)
persistent move_state
if isempty(move_state),move_state=zeros(1,22);end
v_ref_cmd=u(2);id_ref_cmd=u(3);iq_test_mode=u(4);iq_test_ref=u(5);Position_Loop_EN=u(6);Close_Loop_EN=u(7);PWM_EN=u(8);PI_Reset_EN=u(9);
if u(10)~=0,v_ref_cmd=replay(1);PWM_EN=replay(2);PI_Reset_EN=replay(3);end
cfg=[Ts_ACR Ts_POS Host_Start_s Host_Traj_Vmax Host_Traj_Amax Host_Traj_Jmax Host_Speed_Ramp_s Pos_deadband Host_Ready_Ticks Host_AutoStart_EN];
[move_state,x_ref_mm,o]=axu5ev_experiment_point_move_step(move_state,t,x_actual_mm,u(1),u(11),Position_Loop_EN~=0 && Close_Loop_EN~=0 && iq_test_mode==0,PWM_EN,PI_Reset_EN,alignment_enabled,alignment_ready,cfg);
target_accepted_mm=o(1);move_busy=o(2);in_position=o(3);command_status=o(4);segment_start_mm=o(5);segment_start_s=o(6);trajectory_done=o(7);move_ready=o(8);accepted_count=o(9);rejected_count=o(10);segment_id=o(11);command_received_s=o(12);move_interrupted=o(13);
if alignment_enabled~=0 && alignment_ready==0
 Position_Loop_EN=0;Close_Loop_EN=0;iq_test_mode=1;iq_test_ref=0;
end
trajectory_config=[Host_Traj_Vmax Host_Traj_Amax Host_Traj_Jmax Host_Speed_Ramp_s Ts_ACR];
vdc=Udc;load_N=Host_Load_N;
end

function [s,x_ref,obs]=axu5ev_experiment_point_move_step(s,t,x,requested,request_bit,mode_ok,pwm,pi_reset,align_enabled,align_ready,cfg)
%#codegen
% 无隐藏状态：调用者保存s；只接收静止到静止绝对点位。
% cfg: Ts_ACR,Ts_POS,Start,V,A,J,minRamp,deadband,ReadyTicks,AutoStart。
% s: init,lastreq,x0,target,t0,busy,done,inpos,count,status,accepted,rejected,
% interrupted,lasttick,lastref,alignready,unused,duration,received,segment,ready,unused。
if s(1)==0
 s(1)=1;s(2)=request_bit;s(3)=x;s(4)=x;s(5)=t;s(7)=1;s(14)=-1;s(15)=x;s(16)=align_ready;
 if cfg(10)~=0 && align_enabled==0
  s(3)=0;s(4)=requested;s(5)=cfg(3);s(6)=1;s(7)=0;s(10)=1;s(11)=1;s(20)=1;
 end
end
allowed=mode_ok~=0 && pwm~=0 && pi_reset==0 && align_ready~=0;
tick=floor(t/cfg(1)+1e-7);
new_tick=tick~=s(14);
if new_tick
 s(14)=tick;
 if align_enabled~=0 && align_ready~=0 && s(16)==0
  s(3)=x;s(4)=x;s(5)=t;s(6)=0;s(7)=1;s(8)=0;s(9)=0;s(13)=0;s(15)=x;
 end
 s(16)=align_ready;
 if s(6)~=0 && (pwm==0 || pi_reset~=0)
  s(6)=0;s(7)=0;s(8)=0;s(9)=0;s(13)=1;s(10)=7;
 end
end
if s(13)~=0
 x_ref=s(15);
else
 [dx,~,duration]=axu5ev_experiment_scurve_profile(t-s(5),s(4)-s(3),cfg(4),cfg(5),cfg(6),cfg(7));
 x_ref=s(3)+dx;s(18)=duration;s(7)=double(t-s(5)>=duration);
end
% 位置事件与原调度首拍9.9ms对齐；不以速度纹波作为严格零速条件。
if mod(tick,round(cfg(2)/cfg(1)))==round(cfg(2)/cfg(1))-1 && s(22)~=tick+1
 s(22)=tick+1;
 if allowed && s(7)~=0 && s(13)==0 && abs(x-s(4))<=cfg(8)+1e-9
  s(9)=min(s(9)+1,cfg(9));
 else
  s(9)=0;
 end
 s(8)=double(s(9)>=cfg(9));if s(8)~=0,s(6)=0;end
end
s(21)=double(allowed && s(8)~=0 && s(6)==0 && s(13)==0);
if new_tick && ~isequaln(request_bit,s(2))
 s(2)=request_bit;s(19)=t;
 if ~isfinite(requested) || ~isfinite(request_bit) || (request_bit~=0 && request_bit~=1)
  s(10)=4;s(12)=s(12)+1;
 elseif ~allowed
  s(10)=6;s(12)=s(12)+1;
 elseif s(21)==0
  s(10)=3;s(12)=s(12)+1;
 elseif abs(requested-s(4))<=1e-12
  s(10)=5;
 else
  s(3)=s(4);s(4)=requested;s(5)=t;s(6)=1;s(7)=0;s(8)=0;s(9)=0;s(10)=2;s(11)=s(11)+1;s(19)=t;s(20)=s(20)+1;s(21)=0;
  x_ref=s(3);
 end
end
s(15)=x_ref;
obs=[s(4) s(6) s(8) s(10) s(3) s(5) s(7) s(21) s(11) s(12) s(20) s(19) s(13)];
end

function [x,v,T,Ta,Tc] = axu5ev_experiment_scurve_profile(t,target,Vmax,Amax,Jmax,minRamp)
%#codegen
% Smooth velocity ramps with a constant-speed middle segment (mm, seconds).
% Short moves reduce peak velocity; acceleration and jerk remain bounded.
assert(Vmax>0 && Amax>0 && Jmax>0 && minRamp>0);
D=abs(target);x=0;v=0;T=0;Ta=0;Tc=0;
if D==0,return;end
C=10/sqrt(3);
V=min([Vmax,D/minRamp,sqrt(D*Amax/1.875),(D^2*Jmax/C)^(1/3)]);
Ta=max([minRamp,1.875*V/Amax,sqrt(C*V/Jmax)]);
Tc=max(0,D/V-Ta);T=2*Ta+Tc;
if t<=0
 return
elseif t<Ta
 s=t/Ta;
 x=V*Ta*(2.5*s^4-3*s^5+s^6);
 v=V*(10*s^3-15*s^4+6*s^5);
elseif t<Ta+Tc
 x=V*Ta/2+V*(t-Ta);v=V;
elseif t<T
 s=(t-Ta-Tc)/Ta;
 x=V*Ta/2+V*Tc+V*Ta*(s-2.5*s^4+3*s^5-s^6);
 v=V*(1-10*s^3+15*s^4-6*s^5);
else
 x=D;v=0;
end
x=sign(target)*x;v=sign(target)*v;
end
